simulink model "GUAM_uniqueworking"  (R2024b)
settings: Solver=FixedStepAuto  StartTime=0.0  StopTime=SimIn.stopTime  FixedStep=SimIn.Environment.Turbulence.dT  RelTol=1e-6
values from neighbouring files (symbols this model uses):
  SimIn = setup(SimIn, target)    [simSetup.m]
undefined symbols (not defined in the file or in its folder): SimPar
libraries: simulink x1
settings Model: Creator=tbritton  LastModifiedBy=tatiana
settings SolverCC: AlgebraicLoopSolver=TrustRegion
settings DataIOCC: SaveFormat=Structure  SaveOutput=off  DSMLogging=off  SaveTime=off  ReturnWorkspaceOutputs=off
settings OptimizationCC: ReuseModelBlockBuffer=off
settings DebuggingCC: ReadBeforeWriteMsg=DisableAll  WriteAfterWriteMsg=DisableAll  WriteAfterReadMsg=DisableAll  MultiTaskDSMMsg=none  UnconnectedInputMsg=warning  UnconnectedOutputMsg=warning  UnconnectedLineMsg=warning  InitInArrayFormatMsg=none
settings ModelReferenceCC: UpdateModelReferenceTargets=IfOutOfDate  EnableRefExpFcnMdlSchedulingChecks=on
settings SFSimCC: SFSimEcho=off  CustomCodeUndefinedFunction=UseInterfaceOnly
settings RTWCC: GPUComputeCapability=3.5  DLArmComputeVersion=19.05

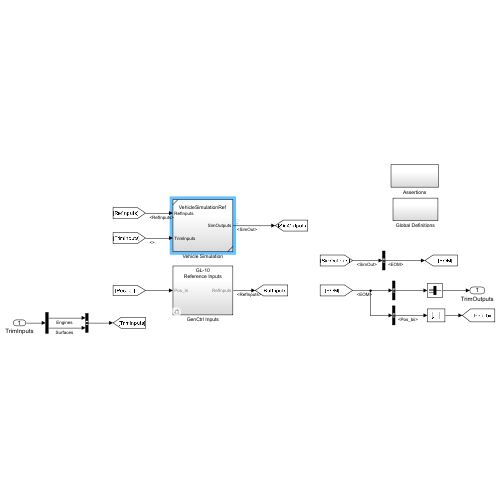
[thumbnail: Simulink's stored preview of the top-level diagram]
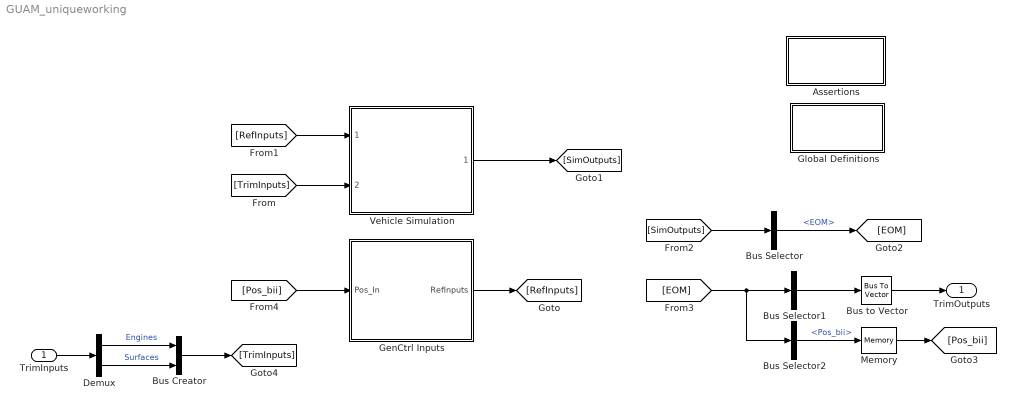
== system GUAM_uniqueworking ==
  TrimInputs : Inport
  Assertions : Subsystem
  Bus Creator : BusCreator  Inputs=2  OutDataTypeStr=Bus: BUS_TRIM_INPUT
  Bus Selector : BusSelector  OutputSignals=Vehicle.EOM
  Bus Selector1 : BusSelector  OutputSignals=AirRelativeData.Veas,AirRelativeData.Vtot,AirRelativeData.alpha,AirRelativeData.beta,WorldRelativeData.gamma,WorldRelativeData.chi,InertialData.Asensed_bIb,AirRelativeData.Vtotdot,AirRelativeData.alphadot,AirRelativeData.betadot,WorldRelativeData.gammadot,WorldRelativeData.chidot,WorldRelativeData.VelDtH_bEh,WorldRelativeData.Euler.phi,WorldRelativeData.Euler.theta,WorldRelativeData.Euler.psi  OutputAsBus=on
  Bus Selector2 : BusSelector  OutputSignals=InertialData.Pos_bii
  Bus to Vector : BusToVector
  Demux : Demux  Outputs=[SimIn.Trim.numEngines SimIn.Trim.numSurfaces]
  GenCtrl Inputs : Subsystem  Variant=on  VariantControl=Variant1
  Global Definitions : Subsystem
  Memory : Memory
  Vehicle Simulation : Subsystem  ReferencedSubsystem=VehicleSimulationRef
  TrimOutputs : Outport  OutDataTypeStr=double  VectorParamsAs1DForOutWhenUnconnected=off
  wires:
  TrimInputs/1 -> Demux/1
  Bus to Vector/1 -> TrimOutputs/1
  Bus Selector1/1 -> Bus to Vector/1
  GenCtrl Inputs/1(RefInputs) -> [RefInputs]
  Vehicle Simulation/1 -> [SimOutputs]
  [TrimInputs] -> Vehicle Simulation/2
  [RefInputs] -> Vehicle Simulation/1
  [SimOutputs] -> Bus Selector/1
  Bus Selector/1 -> [EOM]  "<EOM>"
  Bus Creator/1 -> [TrimInputs]
  Demux/2 -> Bus Creator/2  "Surfaces"
  Demux/1 -> Bus Creator/1  "Engines"
  Bus Selector2/1 -> Memory/1  "<Pos_bii>"
  [EOM] -> Bus Selector1/1, Bus Selector2/1
  [Pos_bii] -> GenCtrl Inputs/1(Pos_In)
  Memory/1 -> [Pos_bii]

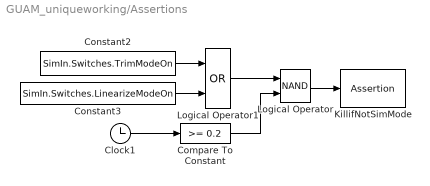
== system GUAM_uniqueworking/Assertions ==
  Clock1 : Clock
  Compare To Constant : simulink/Logic and Bit Operations/Compare To Constant  relop=>=  const=0.2  OutDataTypeStr=boolean  ZeroCross=off
  Constant2 : Constant  Value=SimIn.Switches.TrimModeOn
  Constant3 : Constant  Value=SimIn.Switches.LinearizeModeOn
  KillifNotSimMode : Assertion  AssertionFailFcn="warndlg('Running simulation with TrimMode or LinearizeMode engaged.  Run setup.m to reset.','Warning!')"
  Logical Operator : Logic  Operator=NAND  AllPortsSameDT=off  OutDataTypeStr=boolean
  Logical Operator1 : Logic  Operator=OR  AllPortsSameDT=off  OutDataTypeStr=boolean
  wires:
  Constant2/1 -> Logical Operator1/1
  Compare To Constant/1 -> Logical Operator/2
  Clock1/1 -> Compare To Constant/1
  Logical Operator/1 -> KillifNotSimMode/1
  Constant3/1 -> Logical Operator1/2
  Logical Operator1/1 -> Logical Operator/1

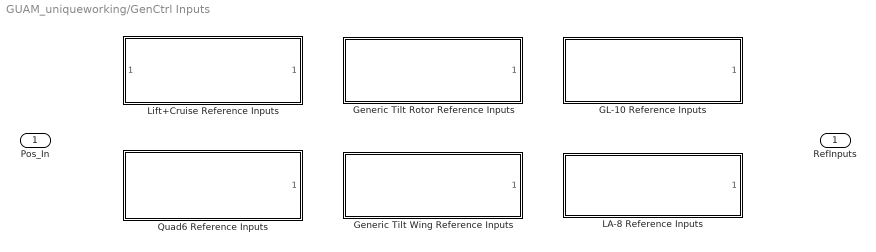
== system GUAM_uniqueworking/GenCtrl Inputs ==
  Pos_In : Inport
  GL-10 Reference Inputs : Subsystem  VariantControl=GVS_VEH_TYPE_GL10  ReferencedSubsystem=GL_10_Reference_Inputs
  Generic Tilt Rotor Reference Inputs : Subsystem  VariantControl=GVS_VEH_TYPE_GTR  ReferencedSubsystem=GTR_Reference_Inputs
  Generic Tilt Wing Reference Inputs : Subsystem  VariantControl=GVS_VEH_TYPE_GTW  ReferencedSubsystem=GTW_Reference_Inputs
  LA-8 Reference Inputs : Subsystem  VariantControl=GVS_VEH_TYPE_LA8  ReferencedSubsystem=LA_8_Reference_Inputs
  Lift+Cruise Reference Inputs : Subsystem  VariantControl=GVS_VEH_TYPE_LC  ReferencedSubsystem=Lift_Cruise_Reference_Inputs
  Quad6 Reference Inputs : Subsystem  VariantControl=GVS_VEH_TYPE_QUAD6  ReferencedSubsystem=Quad6_Reference_Inputs
  RefInputs : Outport  OutDataTypeStr=Bus: BUS_REF_INPUT

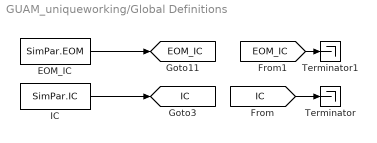
== system GUAM_uniqueworking/Global Definitions ==
  EOM_IC : Constant  Value=SimPar.EOM  OutDataTypeStr=Bus: BUS_PARAM_EOM
  IC : Constant  Value=SimPar.IC  OutDataTypeStr=Bus: BUS_PARAM_IC
  Terminator : Terminator
  Terminator1 : Terminator
  tag scope: EOM_IC=global, IC=global
  wires:
  IC/1 -> [IC]
  EOM_IC/1 -> [EOM_IC]
  [IC] -> Terminator/1
  [EOM_IC] -> Terminator1/1
